simulink model "Track_Mallory_Park_Obstacle_preview"  (R2025a)
settings: Solver=VariableStepAuto  StartTime=0.0  StopTime=100  RelTol=1e-3  EnableMultiTasking=on
libraries: sm_lib x2, nesl_utility x1, sm_car_scene_track_mallory_park_obstacle x1
Description:
  | Copyright 2020-2026 The MathWorks, Inc.
settings Model: Creator=smiller  LastModifiedBy=smiller
settings SolverCC: AlgebraicLoopSolver=TrustRegion
settings DataIOCC: LimitDataPoints=on  ReturnWorkspaceOutputs=off
settings OptimizationCC: ReuseModelBlockBuffer=off  LifeSpan=inf
settings DebuggingCC: UnconnectedInputMsg=warning  UnconnectedOutputMsg=warning  UnconnectedLineMsg=warning  AllowSymbolicDim=off  SFUnexpectedBacktrackingDiag=warning  SFNoUnconditionalDefaultTransitionDiag=warning  SFExecutionAtInitializationDiag=none  ArithmeticOperatorsInVariantConditions=warning
settings ModelReferenceCC: EnableRefExpFcnMdlSchedulingChecks=on
settings SFSimCC: SimUseLocalCustomCode=off  CustomCodeUndefinedFunction=UseInterfaceOnly
settings RTWCC: RTWUseLocalCustomCode=off  GPUComputeCapability=3.5  DLArmComputeVersion=19.05
settings CodeAppCC: StateflowObjectComments=on
settings GRTTargetCC: TargetLangStandard=C89/C90 (ANSI)
settings ConfigComp: CovMetricSettings=dw  CovSaveCumulativeToWorkspaceVar=on  CovSaveSingleToWorkspaceVar=on  CovExternalEMLEnable=off  CovSFcnEnable=off
settings SimscapeCC: SimscapeNominalValues="[{\"value\":\"10\",\"unit\":\"V\"},{\"value\":\"1\",\"unit\":\"A\"},{\"value\":\"10\",\"unit\":\"N*m\"},{\"value\":\"10\",\"unit\":\"bar\"},{\"value\":\"100\",\"unit\":\"kJ/kg\"},{\"value\":\"1\",\"unit\":\"kW\"},{\"value\":\"300\",\"unit\":\"K\"},{\"value\":\"100\",\"unit\":\"cm^3/s\"},{\"value\":\"1\",\"unit\":\"kN\"},{\"value\":\"1\",\"unit\":\"g/cm^3\"},{\"value\":\"1\",\"unit\":\"l\"},{\"value\":\"1\",\"unit\":\"cm^2\"},{\"value\":\"60\",\"unit\":\"Hz\"}]"  SimscapeLogType=all  SimscapeLogDataHistory=10000.0
settings ConfigurationSet: Description=SimMechanics 2G
settings ExplorerConfigSet: InternalSimMechanicsExplorerSettings="<ExplorerConfiguration><canonicalview>default</canonicalview><AnimationSetting><BasePlaybackSpeed>1.0</BasePlaybackSpeed><PlaybackSpeedFactor>8.0</PlaybackSpeedFactor></AnimationSetting><TilePanel><TileInfo><Tiles Columns=\"3\" Count=\"3\" Rows=\"1\"><Column Weight=\"0.2496\"/><Column Weight=\"0.3752\"/><Column Weight=\"0.3752\"/><Row Weight=\"1\"/><Tile Height=\"1\" Width=\"1\" X=\"0\" Y=\"0\"/><Tile Height=\"1\" Width=\"1\" X=\"1\" Y=\"0\"/><Tile Height=\"1\" Width=\"1\" X=\"2\" Y=\"0\"/></Tiles></TileInfo><SceneInfo><SceneViewer><BGColor><R>1</R><G>1</G><B>1</B></BGColor><Camera><DoPerspective>off</DoPerspective><Position><X>-51.106405668965472</X><Y>-45.8533863747829287</Y><Z>454.624922213920172</Z></Position><Center><X>-51.106405668965472</X><Y>-45.8533863747829287</Y><Z>1.47550815143205227</Z></Center><Up><X>-0.997539205676822971</X><Y>0.0701108631928958337</Y><Z>0</Z></Up><ViewLimDist>1</ViewLimDist><YLim>468.011471416423888</YLim><XLim>265.465070343017601</XLim></Camera></SceneViewer><SceneViewer><BGColor><R>1</R><G>1</G><B>1</B></BGColor><Camera><DoPerspective>off</DoPerspective><Position><X>386.776124856355523</X><Y>-375.272836889664063</Y><Z>6.36180498656626181</Z></Position><Center><X>-45.8770168730114989</X><Y>-247.835020843370103</Y><Z>2.55217985239792711</Z></Center><Up><X>-0.00856765321137185551</X><Y>0.000805585008228262844</Y><Z>0.999962972490103907</Z></Up><ViewLimDist>1</ViewLimDist><YLim>4.61417281503467258</YLim><XLim>3.95136346038880815</XLim></Camera></SceneViewer><SceneViewer><BGColor><R>1</R><G>1</G><B>1</B></BGColor><Camera><DoPerspective>off</DoPerspective><Position><X>330.190080728270971</X><Y>-485.927865784491985</Y><Z>49.6611321410396442</Z></Position><Center><X>-38.9084140712043052</X><Y>-232.097879133685524</Y><Z>-3.06732568034722908</Z></Center><Up><X>-0.103085479598772956</X><Y>0.0563940028738164206</Y><Z>0.993072555423700543</Z></Up><ViewLimDist>1</ViewLimDist><YLim>0.623306327282961536</YLim><XLim>0.533770611761652192</XLim></Camera></SceneViewer></SceneInfo></TilePanel><MechEditorPanel><Cameras/><GfxPanelCameraMap/><VideoCreator><PlaybackSpeedRatio>1.0</PlaybackSpeedRatio><FrameRate>30</FrameRate><VideoFormat>Motion JPEG AVI</VideoFormat><FrameSize>auto</FrameSize></VideoCreator></MechEditorPanel></ExplorerConfiguration>"

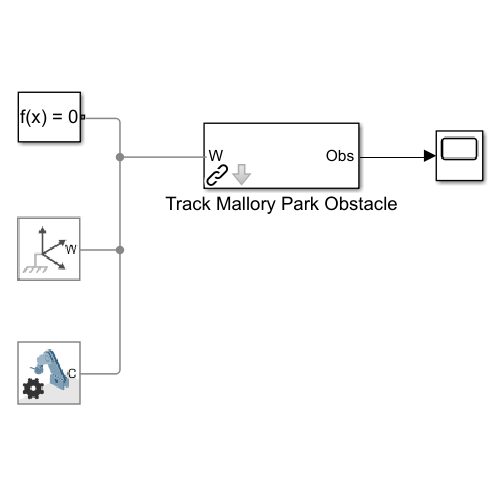
[thumbnail: Simulink's stored preview of the top-level diagram]
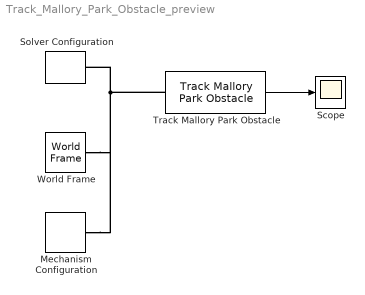
== system Track_Mallory_Park_Obstacle_preview ==
  Mechanism Configuration : sm_lib/Utilities/Mechanism Configuration  UniformGravity=Constant  GravityVector=[0 0 -9.80665]  GravityVectorUnits=m/s^2  LinearizationDelta=0.001  JointModeTransitionNonlinearIterations=2
  Scope : Scope
      settings: ActiveDisplayYMinimum=0.75  ActiveDisplayYMaximum=3.25  DataLoggingSaveFormat=Array
  Solver Configuration : nesl_utility/Solver Configuration  PhysicalDomain=network_engine_domain  SubClassName=solver  LeftPortType=input  RightPortType=generic  Tones=[]  Harmonics=[]  SimulateNoise=off  Profile=off  UseLocalSampling=off  EnableSwitchedLinearOptims=on  FrequencyDomain=off  UseCCode=off  RelTol=0.001  AbsTol=1e-06  MinStep=1e-09  ToWorkspace=off  RevertToSquareIcSolve=off  NumHomotopyIterations=100  PhasorMode=off  PhasorModeNumHarmonics=1  ConsistencySolver=NEWTON_FTOL  IndexReductionMethod=DerivativeReplacement  DoDC=off  ResidualTolerance=1e-09  ConsistencyTolSource=GLOBAL  ConsistencyAbsTol=0.001  ConsistencyRelTol=0.001  ConsistencyTolFactor=0.001  UseLocalSolver=off  LocalSolverChoice=NE_BACKWARD_EULER_ADVANCER  ResolveIndetEquations=on  FunctionEvalNumThread=1  LocalSolverSampleTime=0.001  DoFixedCost=off  MaxNonlinIter=3  MaxModeIter=2  ComputeImpulses=off  ImpulseIterations=2  LinearAlgebra=Sparse  LinearAlgebraNumThread=0  EquationFormulation=NE_TIME_EF  DelaysMemoryBudget=1024  AutomaticFiltering=on  FilteringTimeConstant=0.001  PartitionStorageMethod=AS_NEEDED  PartitionMemoryBudget=1024  PartitionMethod=FAST  MultibodyUseLocalSolver=off  MultibodyLocalSolverChoice=ODE1  MultibodyLocalSolverSampleTime=0.001
  Track Mallory Park Obstacle : sm_car_scene_track_mallory_park_obstacle/Track Mallory Park Obstacle  scene_data=Scene.Mallory_Park_Obstacle
  World Frame : sm_lib/Frames and Transforms/World Frame
  wires:
  Track Mallory Park Obstacle/1 -> Scope/1
  connections:
  Mechanism Configuration/RConn1 -- World Frame/RConn1 -- Track Mallory Park Obstacle/LConn1 -- Solver Configuration/RConn1
